simulink model "lineal_cartpole_sim_OL"  (R2026a)
settings: Solver=ode45  MaxStep=1e-1  RelTol=1e-12  AbsTol=1e-12
undefined symbols (not defined in the file): A, B, C, D
settings Model: Creator=santi  LastModifiedBy=elkin

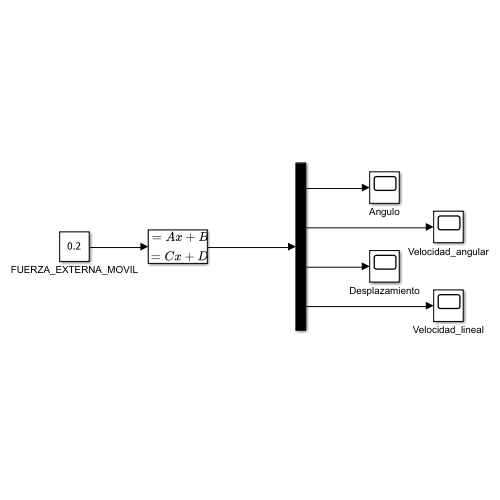
[thumbnail: Simulink's stored preview of the top-level diagram]
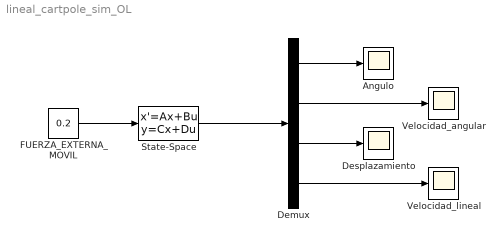
== system lineal_cartpole_sim_OL ==
  Angulo : Scope
      settings: ActiveDisplayYMinimum=-1  ActiveDisplayYMaximum=1
  Demux : Demux
  Desplazamiento : Scope
      settings: ActiveDisplayYMinimum=-1  ActiveDisplayYMaximum=1  DataLoggingVariableName=ScopeData2
  FUERZA_EXTERNA_MOVIL : Constant  Value=0.2
  State-Space : StateSpace  A=A  B=B  C=C  D=D  InitialCondition=[0; 0; 0; 0]
  Velocidad_angular : Scope
      settings: ActiveDisplayYMinimum=-3.3035157546755342E+22  ActiveDisplayYMaximum=2.9731641792079817E+23
  Velocidad_lineal : Scope
      settings: ActiveDisplayYMinimum=-1  ActiveDisplayYMaximum=1  DataLoggingVariableName=ScopeData3
  wires:
  FUERZA_EXTERNA_MOVIL/1 -> State-Space/1
  Demux/1 -> Angulo/1
  Demux/2 -> Velocidad_angular/1
  Demux/3 -> Desplazamiento/1
  Demux/4 -> Velocidad_lineal/1
  State-Space/1 -> Demux/1
